simulink model "CTV_GMEKF"  (R2026a)
settings: Solver=VariableStepAuto
settings Model: DataDictionary=NavigationDictionary.sldd  Creator=David  LastModifiedBy=aparn

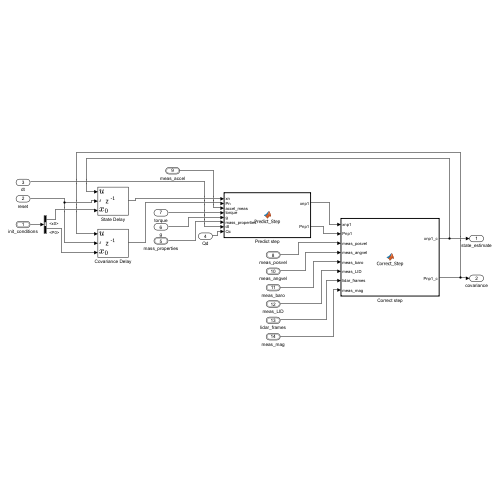
[thumbnail: Simulink's stored preview of the top-level diagram]
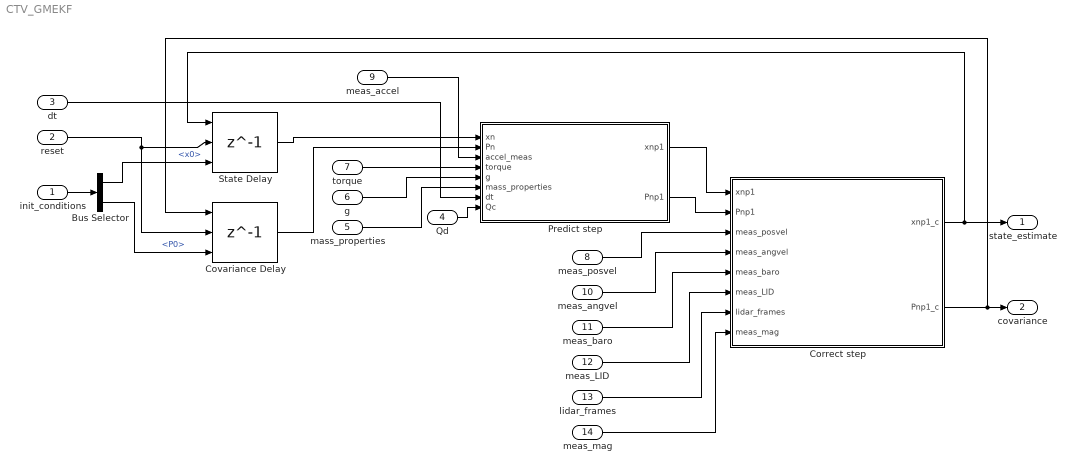
== system CTV_GMEKF ==
  init_conditions : Inport  OutDataTypeStr=Bus: InitConditions
  reset : Inport  Port=2  OutDataTypeStr=ValueType: reset
  dt : Inport  Port=3  OutDataTypeStr=ValueType: timestep
  Qd : Inport  Port=4  OutDataTypeStr=ValueType: Qc
  mass_properties : Inport  Port=5  OutDataTypeStr=Bus: massProperties
  g : Inport  Port=6  OutDataTypeStr=ValueType: gravity
  torque : Inport  Port=7  OutDataTypeStr=ValueType: torque
  meas_posvel : Inport  Port=8  OutDataTypeStr=Bus: gpsBus
  meas_accel : Inport  Port=9  OutDataTypeStr=Bus: accelBus
  meas_angvel : Inport  Port=10  OutDataTypeStr=Bus: angvelBus
  meas_baro : Inport  Port=11  OutDataTypeStr=Bus: baroBus
  meas_LID : Inport  Port=12  OutDataTypeStr=Bus: lidarBus
  lidar_frames : Inport  Port=13  OutDataTypeStr=Bus: lidarFrameBus
  meas_mag : Inport  Port=14  OutDataTypeStr=Bus: magBus
  Bus Selector : BusSelector  OutputSignals=x0,P0
  Correct step : MATLAB Function  TreatAsAtomicUnit=on
  Covariance Delay : Delay  DelayLength=1  InitialConditionSource=Input port  ExternalReset=Rising
      settings: InputPortMap=u0,r5,p4
  Predict step : MATLAB Function  TreatAsAtomicUnit=on
  State Delay : Delay  DelayLength=1  InitialConditionSource=Input port  ExternalReset=Rising
      settings: InputPortMap=u0,r5,p4
  state_estimate : Outport
  covariance : Outport  Port=2
  wires:
  init_conditions/1 -> Bus Selector/1
  Bus Selector/1 -> State Delay/3  "<x0>"
  Bus Selector/2 -> Covariance Delay/3  "<P0>"
  reset/1 -> Covariance Delay/2, State Delay/2
  State Delay/1 -> Predict step/1(xn)
  meas_accel/1 -> Predict step/3(accel_meas)
  dt/1 -> Predict step/7(dt)
  Covariance Delay/1 -> Predict step/2(Pn)
  torque/1 -> Predict step/4(torque)
  g/1 -> Predict step/5(g)
  mass_properties/1 -> Predict step/6(mass_properties)
  Qd/1 -> Predict step/8(Qc)
  Predict step/1(xnp1) -> Correct step/1(xnp1)
  Predict step/2(Pnp1) -> Correct step/2(Pnp1)
  meas_posvel/1 -> Correct step/3(meas_posvel)
  meas_angvel/1 -> Correct step/4(meas_angvel)
  meas_baro/1 -> Correct step/5(meas_baro)
  meas_LID/1 -> Correct step/6(meas_LID)
  lidar_frames/1 -> Correct step/7(lidar_frames)
  meas_mag/1 -> Correct step/8(meas_mag)
  Correct step/2(Pnp1_c) -> Covariance Delay/1, covariance/1
  Correct step/1(xnp1_c) -> State Delay/1, state_estimate/1

== matlab function CTV_GMEKF/Correct step ==
  data: xnp1 input; xnp1_c output; Pnp1 input; meas_posvel input; Pnp1_c output; meas_angvel input; meas_baro input; meas_LID input; lidar_frames input; meas_mag input
function [xnp1_c, Pnp1_c] = Correct_Step(xnp1, Pnp1, meas_posvel, meas_angvel, meas_baro, meas_LID, lidar_frames, meas_mag)
[xnp1_c, Pnp1_c] = gmekf_correct(xnp1, Pnp1, meas_posvel, ...
    meas_angvel, meas_baro, meas_LID, lidar_frames, meas_mag);
end

== matlab function CTV_GMEKF/Predict step ==
  data: xn input; Pn input; xnp1 output; accel_meas input; torque input; g input; mass_properties input; dt input; Pnp1 output; Qc input
function [xnp1, Pnp1] = Predict_Step(xn, Pn, accel_meas, torque, g, mass_properties, dt, Qc)
% Unpack the structs
J = mass_properties.J;
accel = accel_meas.accel;
validity = accel_meas.validity;
[xnp1, Pnp1] = gmekf_predict(xn, Pn, accel, torque, validity, J, g, dt, Qc);
end
